simulink model "Controller"  (R2018b)
settings: configuration reference "control_config" (kept outside this file)
values from neighbouring files (symbols this model uses):
  CONTROL_EXPORT = Simulink.Parameter(CONTROL_EXPORT_VALUE)    [controller_model_init.m]
  CONTROL_PARAM = Simulink.Parameter(CONTROL_PARAM_VALUE)    [controller_model_init.m]
undefined symbols (not defined in the file or in its folder): actuator_cmd, ControlMode, DiscIntNeverNeededParam, timestamp
libraries: simulink x7, FMT_Model_Lib x5
settings Model: Creator=jc  LastModifiedBy=zouji
settings ConfigSetRef: SourceLocation=Base Workspace

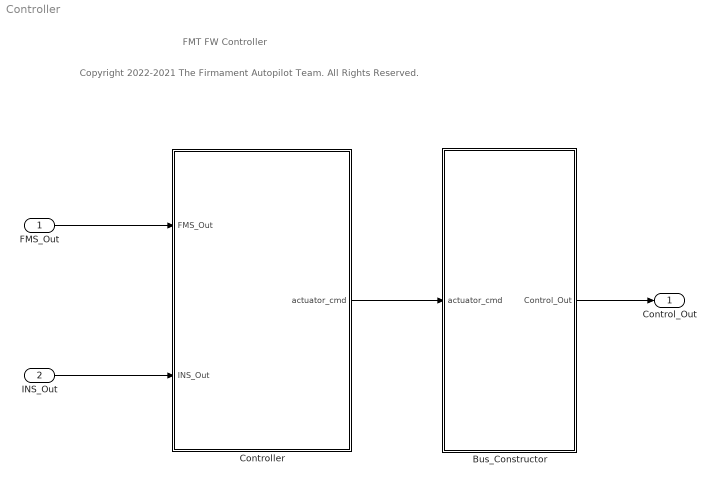
== system Controller ==
  note: Copyright 2022-2021 The Firmament Autopilot Team. All Rights Reserved.
  note: FMT FW Controller
  FMS_Out : Inport  OutDataTypeStr=Bus: FMS_Out_Bus
  INS_Out : Inport  Port=2  OutDataTypeStr=Bus: INS_Out_Bus
  Bus_Constructor : Subsystem
  Controller : Subsystem
  Control_Out : Outport  OutDataTypeStr=Bus: Control_Out_Bus
  wires:
  FMS_Out/1 -> Controller/1(FMS_Out)
  INS_Out/1 -> Controller/2(INS_Out)
  Controller/1(actuator_cmd) -> Bus_Constructor/1(actuator_cmd)
  Bus_Constructor/1(Control_Out) -> Control_Out/1

== system Controller/Bus_Constructor ==
  actuator_cmd : Inport
  Bus Assignment : BusAssignment  AssignedSignals=actuator_cmd,timestamp
  Constant : Constant  Value=0  OutDataTypeStr=Bus: Control_Out_Bus
  timestamp : Subsystem  mask{sample_time=CONTROL_EXPORT.period}
      mask prompts: sample_time "sample time (ms)"
  Control_Out : Outport
  wires:
  actuator_cmd/1 -> Bus Assignment/2
  Constant/1 -> Bus Assignment/1
  Bus Assignment/1 -> Control_Out/1
  timestamp/1(timestamp_ms) -> Bus Assignment/3

== system Controller/Controller ==
  FMS_Out : Inport
  INS_Out : Inport  Port=2
  Airspeed : Subsystem
  Attitude_Control : Subsystem
  Control_Allocation : Subsystem  Variant=on
      settings: GeneratePreprocessorConditionals=on
  Lateral_Control : Subsystem
  Mux : Mux  Inputs=2
  TECS_Core : Subsystem
  actuator_cmd : Outport
  wires:
  INS_Out/1 -> Attitude_Control/3(INS_Out), Lateral_Control/2(INS_Out), TECS_Core/3(INS_Out), Airspeed/1(INS_Out)
  Attitude_Control/1(torque_cmd) -> Control_Allocation/2(torque_cmd)
  TECS_Core/2(throttle_cmd) -> Control_Allocation/3(line_acc_cmd)
  Lateral_Control/1(phi_cmd) -> TECS_Core/1(pos_phi_cmd), Mux/1
  TECS_Core/1(theta_cmd) -> Mux/2
  Mux/1 -> Attitude_Control/4(att_cmd)
  Control_Allocation/1(actuator_cmd) -> actuator_cmd/1
  FMS_Out/1 -> TECS_Core/2(FMS_Out), Lateral_Control/1(FMS_Out), Control_Allocation/1(FMS_Out), Attitude_Control/1(FMS_Out)
  Airspeed/1(Vt) -> Attitude_Control/2(Vt), TECS_Core/4(Vt)

== system Controller/Bus_Constructor/timestamp ==
  Constant : Constant  Value=sample_time
  Data Type Conversion : DataTypeConversion  OutDataTypeStr=uint32
  Discrete-Time Integrator : DiscreteIntegrator  IntegratorMethod=Accumulation: Forward Euler  SampleTime=-1  ICPrevOutput=DiscIntNeverNeededParam  ICPrevScaledInput=DiscIntNeverNeededParam
  timestamp_ms : Outport
  wires:
  Discrete-Time Integrator/1 -> Data Type Conversion/1
  Constant/1 -> Discrete-Time Integrator/1
  Data Type Conversion/1 -> timestamp_ms/1

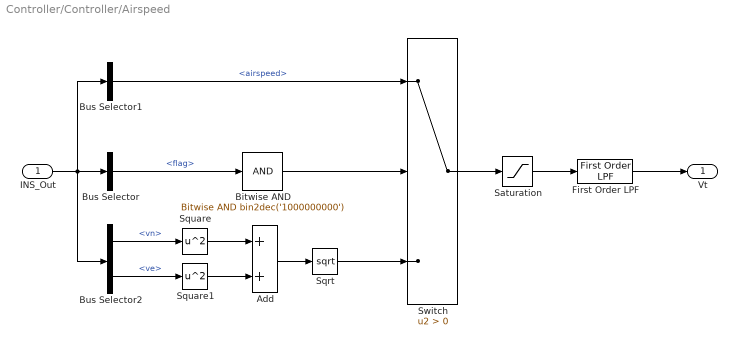
== system Controller/Controller/Airspeed ==
  INS_Out : Inport
  Add : Sum
  Bitwise AND : simulink/Logic and Bit Operations/Bitwise Operator  logicop=AND  UseBitMask=on  BitMask=bin2dec('1000000000')  BitMaskRealWorld=Stored Integer
  Bus Selector : BusSelector  OutputSignals=flag
  Bus Selector1 : BusSelector  OutputSignals=airspeed
  Bus Selector2 : BusSelector  OutputSignals=vn,ve
  First Order LPF : FMT_Model_Lib/Filter/First Order LPF  fc=20
      settings: SourceProductName=FMT Toolbox
  Saturation : Saturate  UpperLimit=100  LowerLimit=0.1
  Sqrt : Sqrt  SaturateOnIntegerOverflow=on
  Square : Math  Operator=square  SaturateOnIntegerOverflow=on
  Square1 : Math  Operator=square  SaturateOnIntegerOverflow=on
  Switch : Switch  Criteria=u2 > Threshold
  Vt : Outport
  wires:
  INS_Out/1 -> Bus Selector2/1, Bus Selector1/1, Bus Selector/1
  Bitwise AND/1 -> Switch/2
  Bus Selector/1 -> Bitwise AND/1  "<flag>"
  Bus Selector1/1 -> Switch/1  "<airspeed>"
  Bus Selector2/1 -> Square/1  "<vn>"
  Bus Selector2/2 -> Square1/1  "<ve>"
  Square/1 -> Add/1
  Square1/1 -> Add/2
  Add/1 -> Sqrt/1
  Sqrt/1 -> Switch/3
  Switch/1 -> Saturation/1
  Saturation/1 -> First Order LPF/1
  First Order LPF/1 -> Vt/1

== system Controller/Controller/Attitude_Control ==
  FMS_Out : Inport
  Vt : Inport  Port=2
  INS_Out : Inport  Port=3
  att_cmd : Inport  Port=4
  Innerloop_Rate_Control : Subsystem
  Outloop_Angle_Control : Subsystem
  torque_cmd : Outport
  wires:
  INS_Out/1 -> Innerloop_Rate_Control/3(INS_Out), Outloop_Angle_Control/2(INS_Out)
  FMS_Out/1 -> Innerloop_Rate_Control/2(FMS_Out), Outloop_Angle_Control/3(FMS_Out)
  Outloop_Angle_Control/1(euler_rate_cmd) -> Innerloop_Rate_Control/1(euler_rate_cmd)
  Innerloop_Rate_Control/1(rate_dot_cmd) -> torque_cmd/1
  att_cmd/1 -> Outloop_Angle_Control/1(att_cmd)
  Vt/1 -> Innerloop_Rate_Control/4(Vt), Outloop_Angle_Control/4(Vt)

== system Controller/Controller/Control_Allocation ==
  note: 1) Add Subsystem or Model blocks as valid variant choices.
      | 2) You cannot connect blocks at this level. At simulation, connectivity is automatically
      | determined, based on the active variant and port name matching.
  FMS_Out : Inport
  torque_cmd : Inport  Port=2
  line_acc_cmd : Inport  Port=3
  Fixwing : Subsystem  TreatAsAtomicUnit=on  VariantControl=AIRFRAME==1
      mask Display: image('.\figures\fixwing.png');
  actuator_cmd : Outport

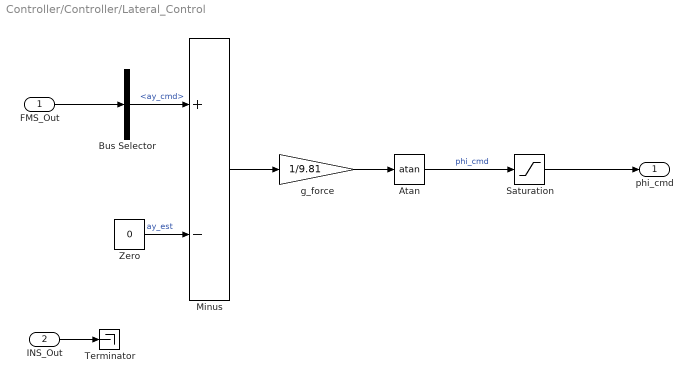
== system Controller/Controller/Lateral_Control ==
  FMS_Out : Inport
  INS_Out : Inport  Port=2
  Atan : Trigonometry  Operator=atan
  Bus Selector : BusSelector  OutputSignals=ay_cmd
  Minus : Sum  Inputs=+-
  Saturation : Saturate  UpperLimit=CONTROL_PARAM.ROLL_PITCH_CMD_LIM  LowerLimit=-CONTROL_PARAM.ROLL_PITCH_CMD_LIM
  Terminator : Terminator
  Zero : Constant  Value=0  OutDataTypeStr=Inherit: Inherit via back propagation
  g_force : Gain  Gain=1/9.81
  phi_cmd : Outport
  wires:
  FMS_Out/1 -> Bus Selector/1
  Bus Selector/1 -> Minus/1  "<ay_cmd>"
  Zero/1 -> Minus/2  "ay_est"
  Minus/1 -> g_force/1
  g_force/1 -> Atan/1
  Atan/1 -> Saturation/1  "phi_cmd"
  INS_Out/1 -> Terminator/1
  Saturation/1 -> phi_cmd/1

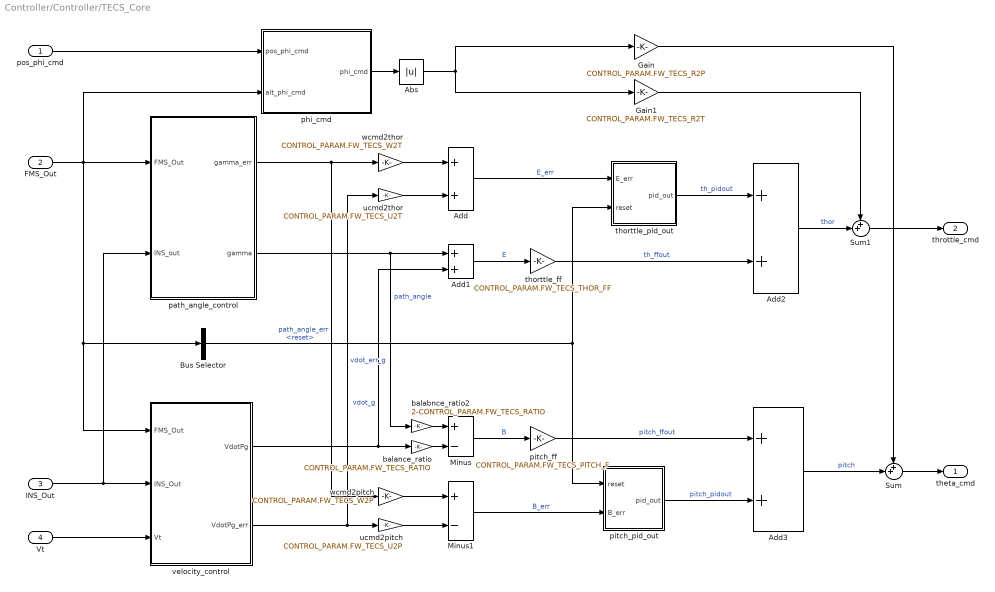
== system Controller/Controller/TECS_Core ==
  pos_phi_cmd : Inport
  FMS_Out : Inport  Port=2
  INS_Out : Inport  Port=3
  Vt : Inport  Port=4
  Abs : Abs
  Add{,1..3} (4 alike) : Sum
  Bus Selector : BusSelector  OutputSignals=reset
  Gain : Gain  Gain=CONTROL_PARAM.FW_TECS_R2P
  Gain1 : Gain  Gain=CONTROL_PARAM.FW_TECS_R2T
  Minus : Sum  Inputs=+-
  Minus1 : Sum  Inputs=+-
  Sum : Sum  Inputs=++|
  Sum1 : Sum  Inputs=++|
  balabnce_ratio2 : Gain  Gain=2-CONTROL_PARAM.FW_TECS_RATIO
  balance_ratio : Gain  Gain=CONTROL_PARAM.FW_TECS_RATIO
  path_angle_control : Subsystem
  phi_cmd : Subsystem
  pitch_ff : Gain  Gain=CONTROL_PARAM.FW_TECS_PITCH_F
  pitch_pid_out : Subsystem
  thorttle_ff : Gain  Gain=CONTROL_PARAM.FW_TECS_THOR_FF
  thorttle_pid_out : Subsystem
  ucmd2pitch : Gain  Gain=CONTROL_PARAM.FW_TECS_U2P
  ucmd2thor : Gain  Gain=CONTROL_PARAM.FW_TECS_U2T
  velocity_control : Subsystem
  wcmd2pitch : Gain  Gain=CONTROL_PARAM.FW_TECS_W2P
  wcmd2thor : Gain  Gain=CONTROL_PARAM.FW_TECS_W2T
  theta_cmd : Outport
  throttle_cmd : Outport  Port=2
  wires:
  INS_Out/1 -> path_angle_control/2(INS_out), velocity_control/2(INS_Out)
  path_angle_control/1(gamma_err) -> wcmd2pitch/1, wcmd2thor/1  "path_angle_err"
  velocity_control/2(VdotPg_err) -> ucmd2thor/1, ucmd2pitch/1  "vdot_err_g"
  velocity_control/1(VdotPg) -> Add1/2, balance_ratio/1  "vdot_g"
  path_angle_control/2(gamma) -> balabnce_ratio2/1, Add1/1  "path_angle"
  Minus/1 -> pitch_ff/1  "B"
  Add1/1 -> thorttle_ff/1  "E"
  thorttle_ff/1 -> Add2/2  "th_ffout"
  Bus Selector/1 -> pitch_pid_out/1(reset), thorttle_pid_out/2(reset)  "<reset>"
  pitch_ff/1 -> Add3/1  "pitch_ffout"
  Add/1 -> thorttle_pid_out/1(E_err)  "E_err"
  thorttle_pid_out/1(pid_out) -> Add2/1  "th_pidout"
  Minus1/1 -> pitch_pid_out/2(B_err)  "B_err"
  pitch_pid_out/1(pid_out) -> Add3/2  "pitch_pidout"
  balabnce_ratio2/1 -> Minus/1
  wcmd2thor/1 -> Add/1
  ucmd2thor/1 -> Add/2
  FMS_Out/1 -> Bus Selector/1, velocity_control/1(FMS_Out), path_angle_control/1(FMS_Out), phi_cmd/2(alt_phi_cmd)
  Sum/1 -> theta_cmd/1
  Sum1/1 -> throttle_cmd/1
  Add2/1 -> Sum1/2  "thor"
  Gain1/1 -> Sum1/1
  pos_phi_cmd/1 -> phi_cmd/1(pos_phi_cmd)
  phi_cmd/1(phi_cmd) -> Abs/1
  wcmd2pitch/1 -> Minus1/1
  ucmd2pitch/1 -> Minus1/2
  Gain/1 -> Sum/1
  Add3/1 -> Sum/2  "pitch"
  Abs/1 -> Gain/1, Gain1/1
  Vt/1 -> velocity_control/3(Vt)
  balance_ratio/1 -> Minus/2

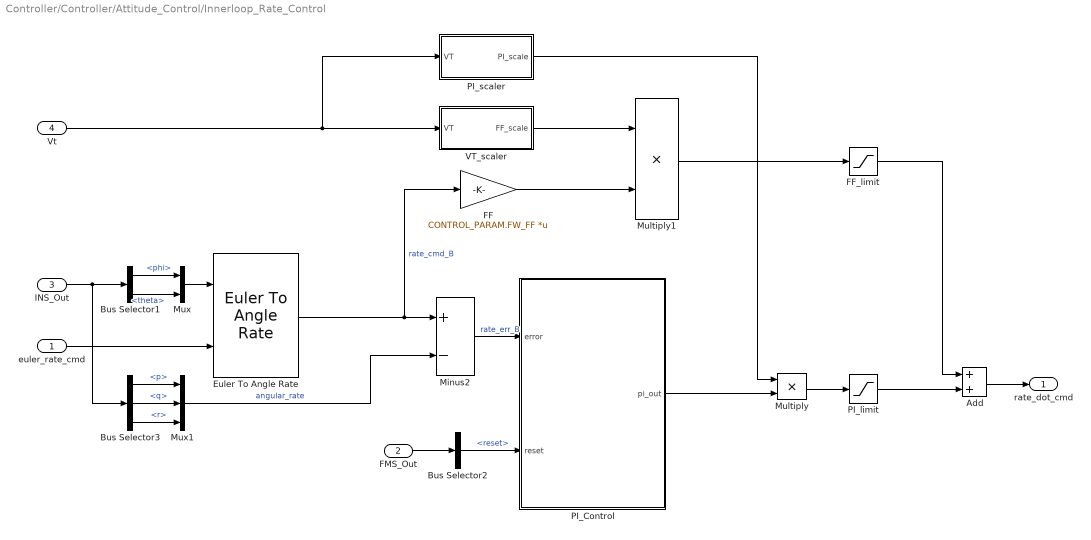
== system Controller/Controller/Attitude_Control/Innerloop_Rate_Control ==
  euler_rate_cmd : Inport
  FMS_Out : Inport  Port=2
  INS_Out : Inport  Port=3
  Vt : Inport  Port=4
  Add : Sum
  Bus Selector1 : BusSelector  OutputSignals=phi,theta
  Bus Selector2 : BusSelector  OutputSignals=reset
  Bus Selector3 : BusSelector  OutputSignals=p,q,r
  Euler To Angle Rate : FMT_Model_Lib/Math/Euler To Angle Rate
      settings: SourceProductName=FMT Toolbox
  FF : Gain  Gain=CONTROL_PARAM.FW_FF  Multiplication=Matrix(K*u)
  FF_limit : Saturate  UpperLimit=CONTROL_PARAM.FW_FF_LIMIT  LowerLimit=-CONTROL_PARAM.FW_FF_LIMIT  OutDataTypeStr=single
  Minus2 : Sum  Inputs=+-
  Multiply : Product
  Multiply1 : Product
  Mux : Mux  Inputs=2
  Mux1 : Mux  Inputs=3
  PI_Control : Subsystem
  PI_limit : Saturate  UpperLimit=CONTROL_PARAM.FW_PI_LIMIT  LowerLimit=-CONTROL_PARAM.FW_PI_LIMIT
  PI_scaler : Subsystem
  VT_scaler : Subsystem
  rate_dot_cmd : Outport
  wires:
  PI_scaler/1(PI_scale) -> Multiply/1
  Multiply1/1 -> FF_limit/1
  FF/1 -> Multiply1/2
  FF_limit/1 -> Add/1
  VT_scaler/1(FF_scale) -> Multiply1/1
  euler_rate_cmd/1 -> Euler To Angle Rate/2
  Multiply/1 -> PI_limit/1
  Euler To Angle Rate/1 -> FF/1, Minus2/1  "rate_cmd_B"
  Mux1/1 -> Minus2/2  "angular_rate"
  PI_limit/1 -> Add/2
  Add/1 -> rate_dot_cmd/1
  Minus2/1 -> PI_Control/1(error)  "rate_err_B"
  Bus Selector2/1 -> PI_Control/2(reset)  "<reset>"
  PI_Control/1(pi_out) -> Multiply/2
  INS_Out/1 -> Bus Selector3/1, Bus Selector1/1
  Bus Selector1/1 -> Mux/1  "<phi>"
  Bus Selector1/2 -> Mux/2  "<theta>"
  Mux/1 -> Euler To Angle Rate/1
  FMS_Out/1 -> Bus Selector2/1
  Bus Selector3/1 -> Mux1/1  "<p>"
  Bus Selector3/2 -> Mux1/2  "<q>"
  Bus Selector3/3 -> Mux1/3  "<r>"
  Vt/1 -> PI_scaler/1(VT), VT_scaler/1(VT)

== system Controller/Controller/Attitude_Control/Outloop_Angle_Control ==
  att_cmd : Inport
  INS_Out : Inport  Port=2
  FMS_Out : Inport  Port=3
  Vt : Inport  Port=4
  Attitude_Controller : Subsystem
  Heading_Controller : Subsystem
  Mux : Mux  Inputs=2
  Reshape : Reshape  OutputDimensionality=Column vector (2-D)
  Signal_Select : Subsystem
  euler_rate_cmd : Outport
  wires:
  FMS_Out/1 -> Heading_Controller/1(FMS_Out), Signal_Select/2(FMS_Out)
  INS_Out/1 -> Attitude_Controller/2(INS_Out)
  att_cmd/1 -> Signal_Select/1(att_cmd_rad)
  Signal_Select/1(out) -> Attitude_Controller/1(att_cmd)
  Attitude_Controller/1(phi_theta_rate_cmd) -> Mux/1
  Heading_Controller/1(psi_rate_cmd) -> Mux/2
  Mux/1 -> Reshape/1
  Reshape/1 -> euler_rate_cmd/1
  Vt/1 -> Heading_Controller/2(Vt)

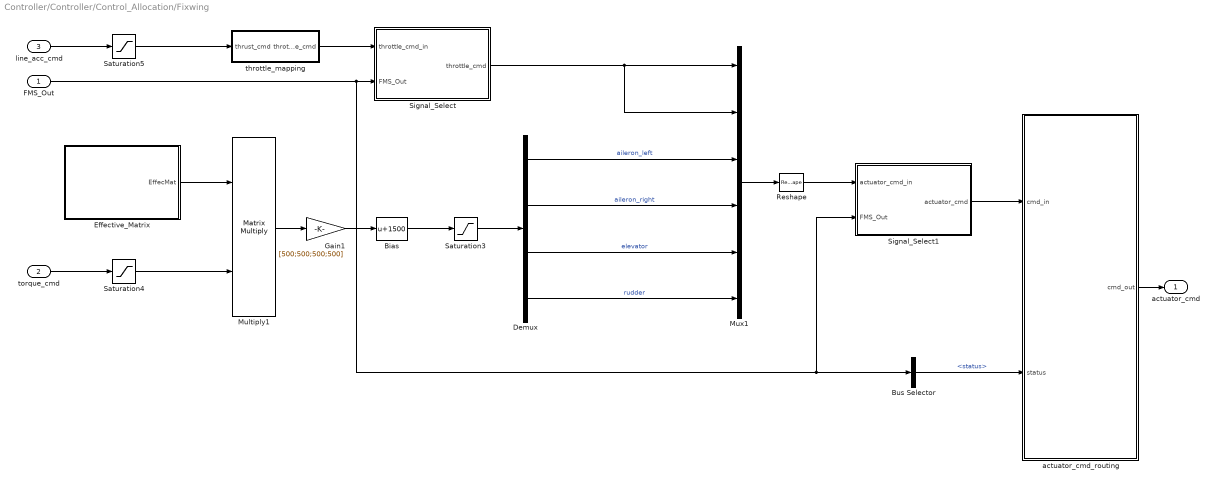
== system Controller/Controller/Control_Allocation/Fixwing ==
  FMS_Out : Inport
  torque_cmd : Inport  Port=2
  line_acc_cmd : Inport  Port=3
  Bias : Bias  Bias=1500
  Bus Selector : BusSelector  OutputSignals=status
  Demux : Demux
  Effective_Matrix : Subsystem
  Gain1 : Gain  Gain=[500;500;500;500]  OutDataTypeStr=Inherit: Same as input  ParamDataTypeStr=Inherit: Same as input
  Multiply1 : Product  Multiplication=Matrix(*)  OutDataTypeStr=Inherit: Same as first input
  Mux1 : Mux  Inputs=6
  Reshape : Reshape  OutputDimensionality=Column vector (2-D)  OutputDimensions=[16,1]
  Saturation3 : Saturate  UpperLimit=2000  LowerLimit=1000  OutDataTypeStr=uint16
  Saturation4 : Saturate  UpperLimit=1  LowerLimit=-1
  Saturation5 : Saturate  UpperLimit=1  LowerLimit=-1
  Signal_Select : Subsystem
  Signal_Select1 : Subsystem
  actuator_cmd_routing : Subsystem
  throttle_mapping : Subsystem
  actuator_cmd : Outport
  wires:
  torque_cmd/1 -> Saturation4/1
  actuator_cmd_routing/1(cmd_out) -> actuator_cmd/1
  Bus Selector/1 -> actuator_cmd_routing/2(status)  "<status>"
  Demux/3 -> Mux1/5  "elevator"
  Demux/1 -> Mux1/3  "aileron_left"
  Saturation4/1 -> Multiply1/2
  Demux/4 -> Mux1/6  "rudder"
  Saturation3/1 -> Demux/1
  Demux/2 -> Mux1/4  "aileron_right"
  Multiply1/1 -> Gain1/1
  Effective_Matrix/1(EffecMat) -> Multiply1/1
  Gain1/1 -> Bias/1
  Saturation5/1 -> throttle_mapping/1(thrust_cmd)
  line_acc_cmd/1 -> Saturation5/1
  Signal_Select/1(throttle_cmd) -> Mux1/2, Mux1/1
  Bias/1 -> Saturation3/1
  throttle_mapping/1(throttle_cmd) -> Signal_Select/1(throttle_cmd_in)
  Mux1/1 -> Reshape/1
  FMS_Out/1 -> Signal_Select/2(FMS_Out), Signal_Select1/2(FMS_Out), Bus Selector/1
  Reshape/1 -> Signal_Select1/1(actuator_cmd_in)
  Signal_Select1/1(actuator_cmd) -> actuator_cmd_routing/1(cmd_in)

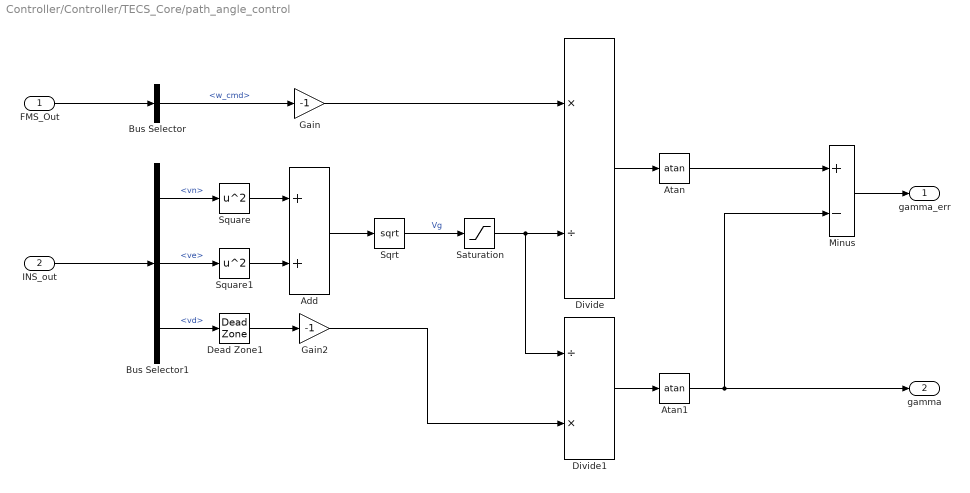
== system Controller/Controller/TECS_Core/path_angle_control ==
  FMS_Out : Inport
  INS_out : Inport  Port=2
  Add : Sum
  Atan : Trigonometry  Operator=atan
  Atan1 : Trigonometry  Operator=atan
  Bus Selector : BusSelector  OutputSignals=w_cmd
  Bus Selector1 : BusSelector  OutputSignals=vn,ve,vd
  Dead Zone1 : DeadZone  LowerValue=-0.1  UpperValue=0.1  SaturateOnIntegerOverflow=on
  Divide : Product  Inputs=*/
  Divide1 : Product  Inputs=/*
  Gain : Gain  Gain=-1
  Gain2 : Gain  Gain=-1
  Minus : Sum  Inputs=+-
  Saturation : Saturate  UpperLimit=100  LowerLimit=8
  Sqrt : Sqrt  SaturateOnIntegerOverflow=on
  Square : Math  Operator=square  SaturateOnIntegerOverflow=on
  Square1 : Math  Operator=square  SaturateOnIntegerOverflow=on
  gamma_err : Outport
  gamma : Outport  Port=2
  wires:
  Atan1/1 -> gamma/1, Minus/2
  Minus/1 -> gamma_err/1
  Atan/1 -> Minus/1
  Sqrt/1 -> Saturation/1  "Vg"
  Add/1 -> Sqrt/1
  Square1/1 -> Add/2
  Square/1 -> Add/1
  Bus Selector1/2 -> Square1/1  "<ve>"
  Bus Selector1/1 -> Square/1  "<vn>"
  Saturation/1 -> Divide1/1, Divide/2
  Gain/1 -> Divide/1
  Divide/1 -> Atan/1
  Bus Selector/1 -> Gain/1  "<w_cmd>"
  FMS_Out/1 -> Bus Selector/1
  Divide1/1 -> Atan1/1
  INS_out/1 -> Bus Selector1/1
  Bus Selector1/3 -> Dead Zone1/1  "<vd>"
  Dead Zone1/1 -> Gain2/1
  Gain2/1 -> Divide1/2

== system Controller/Controller/TECS_Core/phi_cmd ==
  pos_phi_cmd : Inport
  alt_phi_cmd : Inport  Port=2
  Bus Selector1 : BusSelector  OutputSignals=phi_cmd,ctrl_mode
  Compare To Constant : simulink/Logic and Bit Operations/Compare To Constant  relop===  const=uint8([ControlMode.ALTCTL])  OutDataTypeStr=boolean
  Logical Operator : Logic  Operator=OR  Inputs=1  AllPortsSameDT=off  OutDataTypeStr=boolean
  Switch : Switch  Criteria=u2 > Threshold
  phi_cmd : Outport
  wires:
  Bus Selector1/2 -> Compare To Constant/1  "<ctrl_mode>"
  Compare To Constant/1 -> Logical Operator/1
  Logical Operator/1 -> Switch/2
  Bus Selector1/1 -> Switch/1  "<phi_cmd>"
  Switch/1 -> phi_cmd/1  "phi_cmd"
  pos_phi_cmd/1 -> Switch/3
  alt_phi_cmd/1 -> Bus Selector1/1

== system Controller/Controller/TECS_Core/pitch_pid_out ==
  reset : Inport
  B_err : Inport  Port=2
  Add : Sum  Inputs=+++
  D_control : Subsystem
  I_control : Subsystem
  P_control : Gain  Gain=CONTROL_PARAM.FW_TECS_PITCH_P
  Saturation1 : Saturate  UpperLimit=0.3  LowerLimit=-0.3
  pid_out : Outport
  wires:
  B_err/1 -> P_control/1, D_control/1(err), I_control/1(err)
  reset/1 -> I_control/2(reset), D_control/2(reset)
  Add/1 -> pid_out/1
  D_control/1(d_out) -> Saturation1/1
  P_control/1 -> Add/1  "pitch_pout"
  Saturation1/1 -> Add/3  "pitch_dout"
  I_control/1(i_out) -> Add/2  "pitch_iout"

== system Controller/Controller/TECS_Core/thorttle_pid_out ==
  E_err : Inport
  reset : Inport  Port=2
  Add4 : Sum  Inputs=+++
  D_control : Subsystem
  I_control : Subsystem
  P_control : Gain  Gain=CONTROL_PARAM.FW_TECS_THOR_P
  Saturation1 : Saturate  UpperLimit=0.3  LowerLimit=-0.3
  pid_out : Outport
  wires:
  E_err/1 -> P_control/1, D_control/1(err), I_control/1(E_err)
  Add4/1 -> pid_out/1
  reset/1 -> I_control/2(reset), D_control/2(reset)
  D_control/1(D_out) -> Saturation1/1
  P_control/1 -> Add4/1  "th_pout"
  I_control/1(i_out) -> Add4/2  "th_iout"
  Saturation1/1 -> Add4/3  "th_dout"

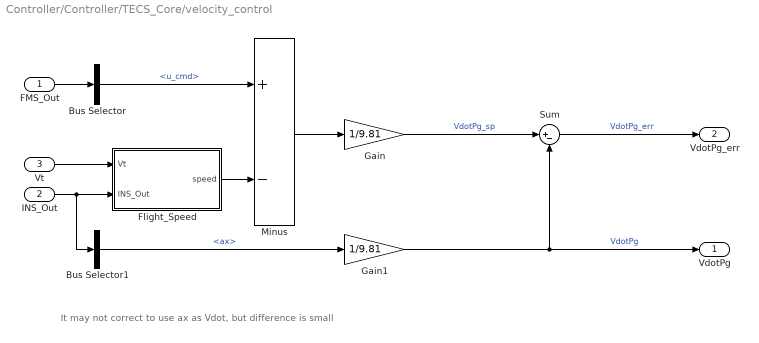
== system Controller/Controller/TECS_Core/velocity_control ==
  note: It may not correct to use ax as Vdot, but difference is small
  FMS_Out : Inport
  INS_Out : Inport  Port=2
  Vt : Inport  Port=3
  Bus Selector : BusSelector  OutputSignals=u_cmd
  Bus Selector1 : BusSelector  OutputSignals=ax
  Flight_Speed : Subsystem
  Gain : Gain  Gain=1/9.81
  Gain1 : Gain  Gain=1/9.81
  Minus : Sum  Inputs=+-
  Sum : Sum  Inputs=|+-
  VdotPg : Outport
  VdotPg_err : Outport  Port=2
  wires:
  FMS_Out/1 -> Bus Selector/1
  Gain1/1 -> Sum/2, VdotPg/1  "VdotPg"
  Bus Selector/1 -> Minus/1  "<u_cmd>"
  Gain/1 -> Sum/1  "VdotPg_sp"
  Minus/1 -> Gain/1
  Sum/1 -> VdotPg_err/1  "VdotPg_err"
  INS_Out/1 -> Bus Selector1/1, Flight_Speed/2(INS_Out)
  Bus Selector1/1 -> Gain1/1  "<ax>"
  Flight_Speed/1(speed) -> Minus/2
  Vt/1 -> Flight_Speed/1(Vt)

== system Controller/Controller/Attitude_Control/Innerloop_Rate_Control/PI_Control ==
  error : Inport
  reset : Inport  Port=2
  Add1 : Sum
  I_Control : Subsystem  mask{p_ki=CONTROL_PARAM.ROLL_RATE_I, q_ki=CONTROL_PARAM.PITCH_RATE_I, r_ki=CONTROL_PARAM.YAW_RATE_I, max_i=CONTROL_PARAM.RATE_I_MAX, min_i=CONTROL_PARAM.RATE_I_MIN}
  P_Control : Subsystem  mask{p_kp=CONTROL_PARAM.ROLL_RATE_P, q_kp=CONTROL_PARAM.PITCH_RATE_P, r_kp=CONTROL_PARAM.YAW_RATE_P}
  pi_out : Outport
  wires:
  Add1/1 -> pi_out/1
  I_Control/1(i_out) -> Add1/2  "i_out"
  error/1 -> P_Control/1(err), I_Control/1(err)
  P_Control/1(p_out) -> Add1/1
  reset/1 -> I_Control/2(reset)

== system Controller/Controller/Attitude_Control/Innerloop_Rate_Control/PI_scaler ==
  VT : Inport
  Divide : Product  Inputs=*/
  Saturation : Saturate  UpperLimit=1  LowerLimit=0
  Square : Math  Operator=square  SaturateOnIntegerOverflow=on
  Square1 : Math  Operator=square  SaturateOnIntegerOverflow=on
  trim_speed : Constant  Value=CONTROL_PARAM.FW_AIRSPEED_TRIM
  PI_scale : Outport
  wires:
  Square1/1 -> Divide/2
  trim_speed/1 -> Square/1
  Square/1 -> Divide/1
  VT/1 -> Square1/1
  Divide/1 -> Saturation/1
  Saturation/1 -> PI_scale/1

== system Controller/Controller/Attitude_Control/Innerloop_Rate_Control/VT_scaler ==
  VT : Inport
  Divide : Product  Inputs=*/
  Saturation : Saturate  UpperLimit=1  LowerLimit=0
  trim_speed : Constant  Value=CONTROL_PARAM.FW_AIRSPEED_TRIM
  FF_scale : Outport
  wires:
  trim_speed/1 -> Divide/1
  VT/1 -> Divide/2
  Divide/1 -> Saturation/1
  Saturation/1 -> FF_scale/1

== system Controller/Controller/Attitude_Control/Outloop_Angle_Control/Attitude_Controller ==
  att_cmd : Inport
  INS_Out : Inport  Port=2
  Error : Subsystem
  P_Controller : Subsystem
  phi_theta_rate_cmd : Outport
  wires:
  INS_Out/1 -> Error/2(INS_Out)
  P_Controller/1(u) -> phi_theta_rate_cmd/1
  att_cmd/1 -> Error/1(att_cmd)
  Error/1(euler_err_rad) -> P_Controller/1(error)

== system Controller/Controller/Attitude_Control/Outloop_Angle_Control/Heading_Controller ==
  FMS_Out : Inport
  Vt : Inport  Port=2
  Bus Selector : BusSelector  OutputSignals=phi_cmd,theta_cmd
  Bus Selector2 : BusSelector  OutputSignals=psi_rate_cmd
  Sum : Sum  Inputs=++|
  Turning_Coordination : Subsystem
  psi_rate_cmd : Outport
  wires:
  Turning_Coordination/1(psi_rate_sp) -> Sum/2
  Sum/1 -> psi_rate_cmd/1
  FMS_Out/1 -> Bus Selector2/1, Bus Selector/1
  Bus Selector/1 -> Turning_Coordination/1(phi_sp)  "<phi_cmd>"
  Bus Selector/2 -> Turning_Coordination/2(theta_sp)  "<theta_cmd>"
  Bus Selector2/1 -> Sum/1  "<psi_rate_cmd>"
  Vt/1 -> Turning_Coordination/3(VT)

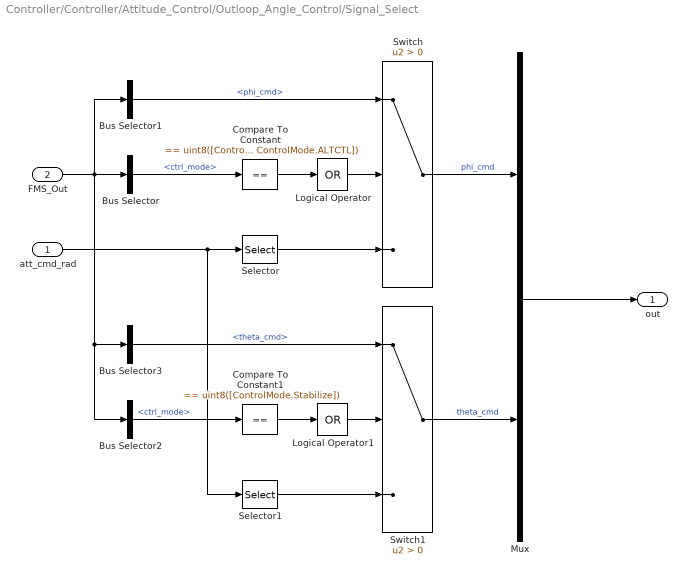
== system Controller/Controller/Attitude_Control/Outloop_Angle_Control/Signal_Select ==
  att_cmd_rad : Inport
  FMS_Out : Inport  Port=2
  Bus Selector : BusSelector  OutputSignals=ctrl_mode
  Bus Selector1 : BusSelector  OutputSignals=phi_cmd
  Bus Selector2 : BusSelector  OutputSignals=ctrl_mode
  Bus Selector3 : BusSelector  OutputSignals=theta_cmd
  Compare To Constant : simulink/Logic and Bit Operations/Compare To Constant  relop===  const=uint8([ControlMode.Stabilize, ControlMode.ALTCTL])  OutDataTypeStr=boolean
  Compare To Constant1 : simulink/Logic and Bit Operations/Compare To Constant  relop===  const=uint8([ControlMode.Stabilize])  OutDataTypeStr=boolean
  Logical Operator : Logic  Operator=OR  Inputs=1  AllPortsSameDT=off  OutDataTypeStr=boolean
  Logical Operator1 : Logic  Operator=OR  Inputs=1  AllPortsSameDT=off  OutDataTypeStr=boolean
  Mux : Mux  Inputs=2
  Selector : Selector  InputPortWidth=2  IndexOptions=Index vector (dialog)  Indices=1  OutputSizes=1
  Selector1 : Selector  InputPortWidth=2  IndexOptions=Index vector (dialog)  Indices=2  OutputSizes=1
  Switch : Switch  Criteria=u2 > Threshold
  Switch1 : Switch  Criteria=u2 > Threshold
  out : Outport
  wires:
  Compare To Constant/1 -> Logical Operator/1
  att_cmd_rad/1 -> Selector/1, Selector1/1
  Bus Selector/1 -> Compare To Constant/1  "<ctrl_mode>"
  FMS_Out/1 -> Bus Selector2/1, Bus Selector3/1, Bus Selector1/1, Bus Selector/1
  Bus Selector1/1 -> Switch/1  "<phi_cmd>"
  Logical Operator/1 -> Switch/2
  Selector/1 -> Switch/3
  Logical Operator1/1 -> Switch1/2
  Compare To Constant1/1 -> Logical Operator1/1
  Bus Selector2/1 -> Compare To Constant1/1  "<ctrl_mode>"
  Bus Selector3/1 -> Switch1/1  "<theta_cmd>"
  Selector1/1 -> Switch1/3
  Switch/1 -> Mux/1  "phi_cmd"
  Switch1/1 -> Mux/2  "theta_cmd"
  Mux/1 -> out/1

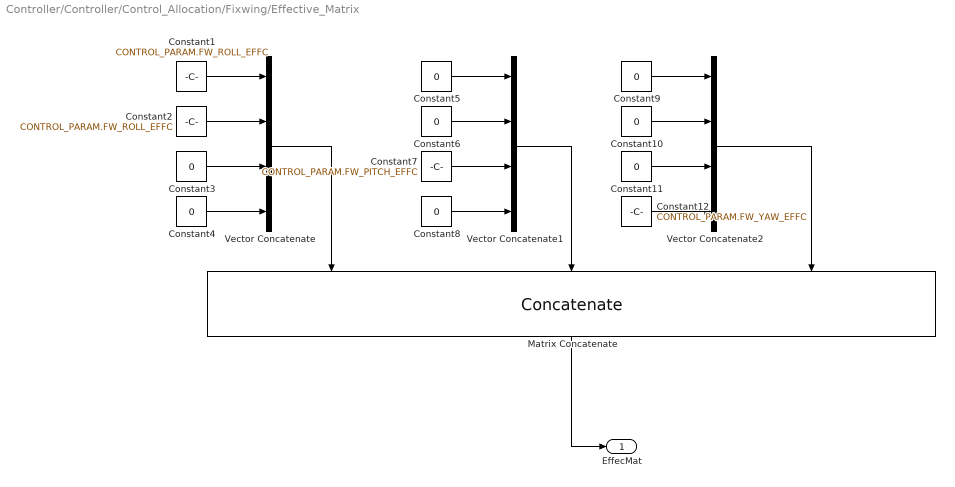
== system Controller/Controller/Control_Allocation/Fixwing/Effective_Matrix ==
  Constant1 : Constant  Value=CONTROL_PARAM.FW_ROLL_EFFC  OutDataTypeStr=single
  Constant{3..6,8..11} (8 alike) : Constant  Value=0  OutDataTypeStr=single
  Constant12 : Constant  Value=CONTROL_PARAM.FW_YAW_EFFC  OutDataTypeStr=single
  Constant2 : Constant  Value=CONTROL_PARAM.FW_ROLL_EFFC  OutDataTypeStr=single
  Constant7 : Constant  Value=CONTROL_PARAM.FW_PITCH_EFFC  OutDataTypeStr=single
  Matrix Concatenate : Concatenate  NumInputs=3  Mode=Multidimensional array  ConcatenateDimension=2
  Vector Concatenate : Concatenate  NumInputs=4
  Vector Concatenate1 : Concatenate  NumInputs=4
  Vector Concatenate2 : Concatenate  NumInputs=4
  EffecMat : Outport
  wires:
  Constant7/1 -> Vector Concatenate1/3
  Constant8/1 -> Vector Concatenate1/4
  Constant9/1 -> Vector Concatenate2/1
  Constant12/1 -> Vector Concatenate2/4
  Constant3/1 -> Vector Concatenate/3
  Vector Concatenate/1 -> Matrix Concatenate/1
  Matrix Concatenate/1 -> EffecMat/1
  Constant2/1 -> Vector Concatenate/2
  Constant11/1 -> Vector Concatenate2/3
  Constant10/1 -> Vector Concatenate2/2
  Constant1/1 -> Vector Concatenate/1
  Vector Concatenate2/1 -> Matrix Concatenate/3
  Constant4/1 -> Vector Concatenate/4
  Vector Concatenate1/1 -> Matrix Concatenate/2
  Constant5/1 -> Vector Concatenate1/1
  Constant6/1 -> Vector Concatenate1/2

== system Controller/Controller/Control_Allocation/Fixwing/Signal_Select ==
  throttle_cmd_in : Inport
  FMS_Out : Inport  Port=2
  Bus Selector1 : BusSelector  OutputSignals=throttle_cmd,ctrl_mode
  Compare To Constant : simulink/Logic and Bit Operations/Compare To Constant  relop===  const=uint8([ControlMode.Manual, ControlMode.Acro, ControlMode.Stabilize])  OutDataTypeStr=boolean
  Logical Operator : Logic  Operator=OR  Inputs=1  AllPortsSameDT=off  OutDataTypeStr=boolean
  Switch : Switch  Criteria=u2 > Threshold
  throttle_cmd : Outport
  wires:
  Logical Operator/1 -> Switch/2
  throttle_cmd_in/1 -> Switch/3
  Switch/1 -> throttle_cmd/1  "throttle_cmd"
  Bus Selector1/2 -> Compare To Constant/1  "<ctrl_mode>"
  Bus Selector1/1 -> Switch/1  "<throttle_cmd>"
  FMS_Out/1 -> Bus Selector1/1
  Compare To Constant/1 -> Logical Operator/1

== system Controller/Controller/Control_Allocation/Fixwing/Signal_Select1 ==
  actuator_cmd_in : Inport
  FMS_Out : Inport  Port=2
  Bus Selector1 : BusSelector  OutputSignals=actuator_cmd,ctrl_mode
  Compare To Constant : simulink/Logic and Bit Operations/Compare To Constant  relop===  const=uint8(ControlMode.Manual)  OutDataTypeStr=boolean
  Selector : Selector  InputPortWidth=16  IndexOptions=Index vector (dialog)  Indices=[1:6]  OutputSizes=1
  Switch : Switch  Criteria=u2 > Threshold
  actuator_cmd : Outport
  wires:
  Compare To Constant/1 -> Switch/2
  actuator_cmd_in/1 -> Switch/3
  Switch/1 -> actuator_cmd/1
  Bus Selector1/2 -> Compare To Constant/1  "<ctrl_mode>"
  Bus Selector1/1 -> Selector/1  "<actuator_cmd>"
  FMS_Out/1 -> Bus Selector1/1
  Selector/1 -> Switch/1

== system Controller/Controller/Control_Allocation/Fixwing/actuator_cmd_routing ==
  cmd_in : Inport
  status : Inport  Port=2
  Constant : Constant  Value=zeros(10,1)  VectorParams1D=off  OutDataTypeStr=uint16
  Disarm : Constant  Value=[1000 1000 1500 1500 1500 1500]'  VectorParams1D=off  OutDataTypeStr=uint16
  Multiport Switch : MultiPortSwitch  DataPortForDefault=Additional data port  DiagnosticForDefault=None
  Mux1 : Mux  Inputs=2
  Reshape : Reshape  OutputDimensionality=Customize  OutputDimensions=[16,1]
  Standby : Constant  Value=[1050 1050 1500 1500 1500 1500]'  VectorParams1D=off  OutDataTypeStr=uint16
  cmd_out : Outport
  wires:
  Disarm/1 -> Multiport Switch/5, Multiport Switch/2
  Reshape/1 -> cmd_out/1
  Constant/1 -> Mux1/2
  Standby/1 -> Multiport Switch/3
  Mux1/1 -> Reshape/1
  status/1 -> Multiport Switch/1
  Multiport Switch/1 -> Mux1/1
  cmd_in/1 -> Multiport Switch/4

== system Controller/Controller/Control_Allocation/Fixwing/throttle_mapping ==
  thrust_cmd : Inport
  Constant1 : Constant  Value=1000  OutDataTypeStr=uint32
  Data Type Conversion : DataTypeConversion  OutDataTypeStr=uint16
  Gain1 : Gain  Gain=1000  OutDataTypeStr=uint32
  Saturation : Saturate  UpperLimit=1  LowerLimit=0
  Sum : Sum  Inputs=|++
  Sum1 : Sum  Inputs=|++
  cruise_throttle : Constant  Value=0.5  OutDataTypeStr=Inherit: Inherit via back propagation
  throttle_cmd : Outport
  wires:
  Sum1/1 -> Data Type Conversion/1
  Saturation/1 -> Gain1/1
  Data Type Conversion/1 -> throttle_cmd/1
  Constant1/1 -> Sum1/2
  Gain1/1 -> Sum1/1
  cruise_throttle/1 -> Sum/2
  Sum/1 -> Saturation/1
  thrust_cmd/1 -> Sum/1

== system Controller/Controller/TECS_Core/pitch_pid_out/D_control ==
  err : Inport
  reset : Inport  Port=2
  DT Filter : FMT_Model_Lib/Filter/DT Filter  fc=10
      settings: SourceProductName=FMT Toolbox
  Gain : Gain  Gain=CONTROL_PARAM.FW_TECS_PITCH_D
  d_out : Outport
  wires:
  reset/1 -> DT Filter/2
  DT Filter/1 -> Gain/1
  Gain/1 -> d_out/1
  err/1 -> DT Filter/1

== system Controller/Controller/TECS_Core/pitch_pid_out/I_control ==
  err : Inport
  reset : Inport  Port=2
  " " : DiscreteIntegrator  ExternalReset=level  InitialConditionSource=external  SampleTime=-1  LimitOutput=on  UpperSaturationLimit=CONTROL_PARAM.FW_TECS_PITCH_I_LIM  LowerSaturationLimit=-CONTROL_PARAM.FW_TECS_PITCH_I_LIM  ICPrevOutput=DiscIntNeverNeededParam  ICPrevScaledInput=DiscIntNeverNeededParam
  Gain3 : Gain  Gain=CONTROL_PARAM.FW_TECS_PITCH_I
  Zero1 : Constant  Value=0  OutDataTypeStr=Inherit: Inherit via back propagation
  i_out : Outport
  wires:
  Zero1/1 -> " "/3
  " "/1 -> i_out/1
  Gain3/1 -> " "/1
  err/1 -> Gain3/1
  reset/1 -> " "/2

== system Controller/Controller/TECS_Core/thorttle_pid_out/D_control ==
  err : Inport
  reset : Inport  Port=2
  DT Filter : FMT_Model_Lib/Filter/DT Filter  fc=30
      settings: SourceProductName=FMT Toolbox
  Gain : Gain  Gain=CONTROL_PARAM.FW_TECS_THOR_D
  D_out : Outport
  wires:
  reset/1 -> DT Filter/2
  DT Filter/1 -> Gain/1
  err/1 -> DT Filter/1
  Gain/1 -> D_out/1

== system Controller/Controller/TECS_Core/thorttle_pid_out/I_control ==
  E_err : Inport
  reset : Inport  Port=2
  " " : DiscreteIntegrator  ExternalReset=level  InitialConditionSource=external  SampleTime=-1  LimitOutput=on  UpperSaturationLimit=CONTROL_PARAM.FW_CRUISE_THRO  LowerSaturationLimit=-CONTROL_PARAM.FW_CRUISE_THRO  ICPrevOutput=DiscIntNeverNeededParam  ICPrevScaledInput=DiscIntNeverNeededParam
  Gain : Gain  Gain=CONTROL_PARAM.FW_TECS_THOR_I
  Zero : Constant  Value=0  OutDataTypeStr=Inherit: Inherit via back propagation
  i_out : Outport
  wires:
  reset/1 -> " "/2
  Zero/1 -> " "/3
  Gain/1 -> " "/1
  E_err/1 -> Gain/1
  " "/1 -> i_out/1

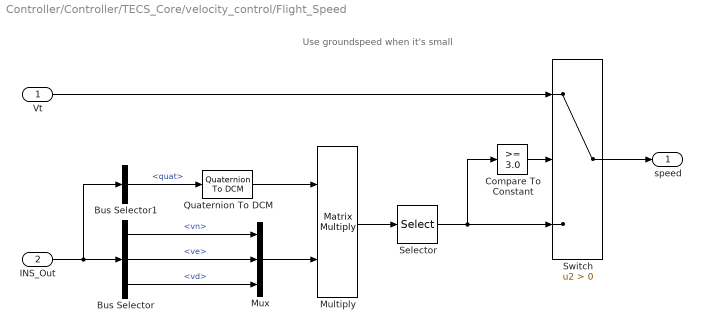
== system Controller/Controller/TECS_Core/velocity_control/Flight_Speed ==
  note: Use groundspeed when it's small
  Vt : Inport
  INS_Out : Inport  Port=2
  Bus Selector : BusSelector  OutputSignals=vn,ve,vd
  Bus Selector1 : BusSelector  OutputSignals=quat
  Compare To Constant : simulink/Logic and Bit Operations/Compare To Constant  relop=>=  const=3.0  OutDataTypeStr=boolean
  Multiply : Product  Multiplication=Matrix(*)
  Mux : Mux  Inputs=3
  Quaternion To DCM : FMT_Model_Lib/Quaternion/Quaternion To DCM
      settings: SourceProductName=FMT Toolbox
  Selector : Selector  InputPortWidth=3  IndexOptions=Index vector (dialog)  Indices=1  OutputSizes=1
  Switch : Switch  Criteria=u2 > Threshold
  speed : Outport
  wires:
  INS_Out/1 -> Bus Selector1/1, Bus Selector/1
  Bus Selector/1 -> Mux/1  "<vn>"
  Bus Selector/2 -> Mux/2  "<ve>"
  Bus Selector/3 -> Mux/3  "<vd>"
  Bus Selector1/1 -> Quaternion To DCM/1  "<quat>"
  Quaternion To DCM/1 -> Multiply/1
  Mux/1 -> Multiply/2
  Multiply/1 -> Selector/1
  Selector/1 -> Compare To Constant/1, Switch/3
  Compare To Constant/1 -> Switch/2
  Vt/1 -> Switch/1
  Switch/1 -> speed/1

== system Controller/Controller/Attitude_Control/Innerloop_Rate_Control/PI_Control/I_Control ==
  err : Inport
  reset : Inport  Port=2
  Constant : Constant  Value=[0;0;0]  OutDataTypeStr=single
  Discrete-Time Integrator : DiscreteIntegrator  ExternalReset=level  InitialConditionSource=external  SampleTime=-1  LimitOutput=on  UpperSaturationLimit=max_i  LowerSaturationLimit=min_i  ICPrevOutput=DiscIntNeverNeededParam  ICPrevScaledInput=DiscIntNeverNeededParam
  Multiply : Product  OutDataTypeStr=Inherit: Same as first input
  Mux : Mux  Inputs=3
  gain1 : Constant  Value=p_ki  OutDataTypeStr=single
  gain2 : Constant  Value=q_ki  OutDataTypeStr=single
  gain3 : Constant  Value=r_ki  OutDataTypeStr=single
  i_out : Outport
  wires:
  err/1 -> Multiply/2
  gain2/1 -> Mux/2
  gain1/1 -> Mux/1
  gain3/1 -> Mux/3
  reset/1 -> Discrete-Time Integrator/2
  Constant/1 -> Discrete-Time Integrator/3
  Discrete-Time Integrator/1 -> i_out/1
  Mux/1 -> Multiply/1
  Multiply/1 -> Discrete-Time Integrator/1

== system Controller/Controller/Attitude_Control/Innerloop_Rate_Control/PI_Control/P_Control ==
  err : Inport
  Multiply : Product  OutDataTypeStr=Inherit: Same as first input
  Mux : Mux  Inputs=3
  gain1 : Constant  Value=p_kp  OutDataTypeStr=single
  gain2 : Constant  Value=q_kp  OutDataTypeStr=single
  gain3 : Constant  Value=r_kp  OutDataTypeStr=single
  p_out : Outport
  wires:
  err/1 -> Multiply/2
  gain2/1 -> Mux/2
  Mux/1 -> Multiply/1
  gain1/1 -> Mux/1
  Multiply/1 -> p_out/1
  gain3/1 -> Mux/3

== system Controller/Controller/Attitude_Control/Outloop_Angle_Control/Attitude_Controller/Error ==
  att_cmd : Inport
  INS_Out : Inport  Port=2
  Bus_Select : Subsystem
  Demux : Demux  Outputs=2
  Mux : Mux  Inputs=2
  Pitch Offset : Bias  Bias=CONTROL_PARAM.FW_PITCH_OFFSET
  Saturation : Saturate  UpperLimit=CONTROL_PARAM.ROLL_PITCH_CMD_LIM  LowerLimit=-CONTROL_PARAM.ROLL_PITCH_CMD_LIM
  Sum : Sum  Inputs=|+-
  euler_err_rad : Outport
  wires:
  att_cmd/1 -> Demux/1  "att_cmd_B_rad"
  Sum/1 -> euler_err_rad/1  "att_error_B_rad"
  INS_Out/1 -> Bus_Select/1(INS_Out)
  Bus_Select/1(att_est_B_rad) -> Sum/2  "att_est_B_rad"
  Demux/2 -> Pitch Offset/1
  Demux/1 -> Mux/1
  Pitch Offset/1 -> Mux/2
  Mux/1 -> Saturation/1
  Saturation/1 -> Sum/1  "att_cmd_B_rad"

== system Controller/Controller/Attitude_Control/Outloop_Angle_Control/Attitude_Controller/P_Controller ==
  error : Inport
  Constant1 : Constant  Value=CONTROL_PARAM.ROLL_P
  Constant2 : Constant  Value=CONTROL_PARAM.PITCH_P
  Multiply : Product
  Mux : Mux  Inputs=2
  u : Outport
  wires:
  Multiply/1 -> u/1
  error/1 -> Multiply/1
  Mux/1 -> Multiply/2
  Constant1/1 -> Mux/1
  Constant2/1 -> Mux/2

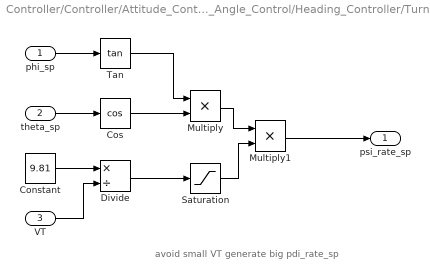
== system Controller/Controller/Attitude_Control/Outloop_Angle_Control/Heading_Controller/Turning_Coordination ==
  note: avoid small VT generate big pdi_rate_sp
  phi_sp : Inport
  theta_sp : Inport  Port=2
  VT : Inport  Port=3
  Constant : Constant  Value=9.81  OutDataTypeStr=single
  Cos : Trigonometry  Operator=cos
  Divide : Product  Inputs=*/
  Multiply : Product
  Multiply1 : Product
  Saturation : Saturate  UpperLimit=1  LowerLimit=0
  Tan : Trigonometry  Operator=tan
  psi_rate_sp : Outport
  wires:
  phi_sp/1 -> Tan/1
  theta_sp/1 -> Cos/1
  Constant/1 -> Divide/1
  VT/1 -> Divide/2
  Tan/1 -> Multiply/1
  Cos/1 -> Multiply/2
  Multiply/1 -> Multiply1/1
  Multiply1/1 -> psi_rate_sp/1
  Divide/1 -> Saturation/1
  Saturation/1 -> Multiply1/2

== system Controller/Controller/Attitude_Control/Outloop_Angle_Control/Attitude_Controller/Error/Bus_Select ==
  INS_Out : Inport
  Bus Selector1 : BusSelector  OutputSignals=phi,theta
  Mux1 : Mux  Inputs=2
  att_est_B_rad : Outport
  wires:
  Bus Selector1/2 -> Mux1/2  "<theta>"
  Bus Selector1/1 -> Mux1/1  "<phi>"
  Mux1/1 -> att_est_B_rad/1
  INS_Out/1 -> Bus Selector1/1
